simulink model "UAV3_Detection_04"  (R2026b)
settings: Solver=FixedStepDiscrete  FixedStep=0.1
settings Model: Creator=Ivan  LastModifiedBy=Ivan

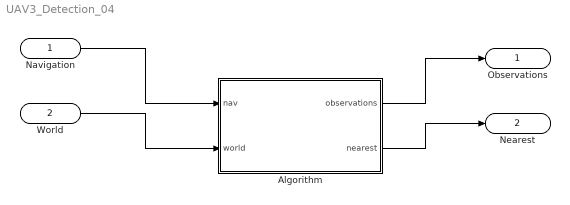
== system UAV3_Detection_04 ==
  Navigation : Inport  OutDataTypeStr=double  PortDimensions=[4 1]
  World : Inport  Port=2  OutDataTypeStr=double  PortDimensions=[3 2]
  Algorithm : MATLAB Function  TreatAsAtomicUnit=on
  Observations : Outport
  Nearest : Outport  Port=2
  wires:
  Navigation/1 -> Algorithm/1(nav)
  World/1 -> Algorithm/2(world)
  Algorithm/1(observations) -> Observations/1
  Algorithm/2(nearest) -> Nearest/1

== matlab function UAV3_Detection_04/Algorithm ==
  data: nav input; observations output; world input; nearest output
function [observations,nearest] = v3_detection(nav,world)
%V3_DETECTION Fixed-size two-obstacle virtual range sensor (35 m).
% world [3x2] = [x;y;radius]. No real optics or computer vision.
% observations [4x2], nearest [boundaryDistance;dx;dy;radius].
%#codegen
observations=zeros(4,2);
nearest=[1000;0;0;0];
for k=1:2
    delta=world(1:2,k)-nav(1:2);
    d=sqrt(sum(delta.^2))-world(3,k);
    if d<=35.0
        observations(:,k)=[world(:,k);1];
        if d<nearest(1)
            nearest=[d;delta(1);delta(2);world(3,k)];
        end
    end
end
end
